simulink model "RESILIENT"  (R2018b)
settings: Solver=VariableStepAuto  StartTime=0.0  StopTime=10.0  RelTol=1e-3
undefined symbols (not defined in the file): sigbuilder_block
settings Model: Creator=lenovo  LastModifiedBy=lenovo

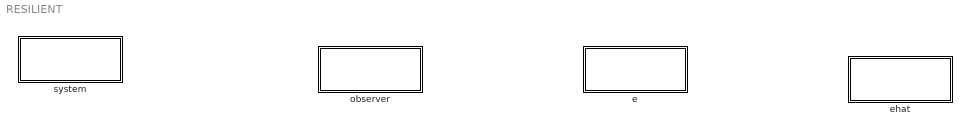
== system RESILIENT ==
  e : Subsystem
  ehat : Subsystem
  observer : Subsystem
  system : Subsystem

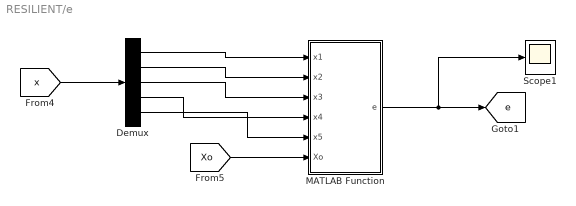
== system RESILIENT/e ==
  Demux : Demux  Outputs=5
  MATLAB Function : MATLAB Function  TreatAsAtomicUnit=on
  Scope1 : Scope
  tag scope: e=global
  wires:
  MATLAB Function/1(e) -> Scope1/1, [e]
  Demux/2 -> MATLAB Function/2(x2)
  Demux/1 -> MATLAB Function/1(x1)
  Demux/5 -> MATLAB Function/5(x5)
  [x] -> Demux/1
  Demux/4 -> MATLAB Function/4(x4)
  [Xo] -> MATLAB Function/6(Xo)
  Demux/3 -> MATLAB Function/3(x3)

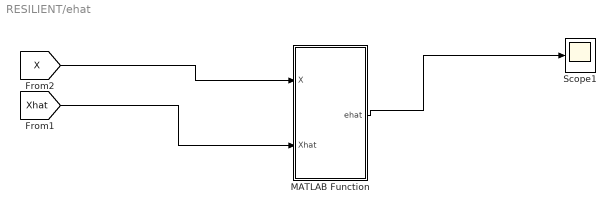
== system RESILIENT/ehat ==
  MATLAB Function : MATLAB Function  TreatAsAtomicUnit=on
  Scope1 : Scope
  wires:
  MATLAB Function/1(ehat) -> Scope1/1
  [X] -> MATLAB Function/1(X)
  [Xhat] -> MATLAB Function/2(Xhat)

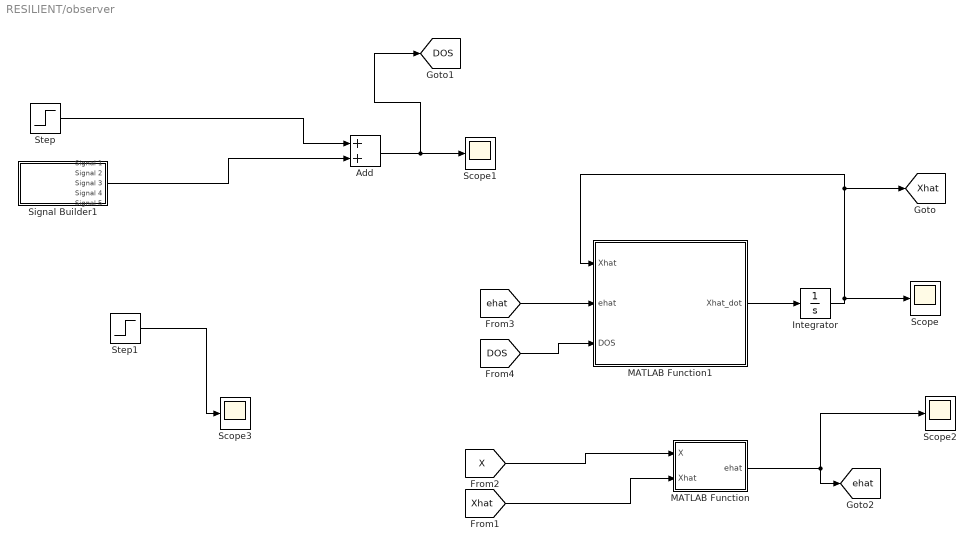
== system RESILIENT/observer ==
  Add : Sum
  Integrator : Integrator  InitialCondition=[-0.5;-1;-1.5;-2;-2.5;-3;-3.5;-4;-4.5;-5;-5.5;-6;0.5;1;1.5;2;2.5;3;3.5;4;4.5;5;5.5;6]
  MATLAB Function : MATLAB Function  TreatAsAtomicUnit=on
  MATLAB Function1 : MATLAB Function  TreatAsAtomicUnit=on
  Scope{,1..3} (4 alike) : Scope
  Signal Builder1 : Subsystem  Tag=STV Subsys  LoadFcn=sigbuilder_block('load',[5.4 30 1141.2 522.6 ]);  StartFcn=sigbuilder_block('start');  StopFcn=sigbuilder_block('stop');  ClipboardFcn=sigbuilder_block('clipboard');  mask(Sigbuilder block){tuvar=[0:10]}
      mask help: Simulink:masks:SigbuilderBlock_MD
      mask init:
      | if ~strcmp(get_param(bdroot(gcbh),'SimulationStatus'),'stopped') tuvar = sigbuilder_block('maskInit'); end
      settings: CopyFcn=sigbuilder_block('copy');  DeleteFcn=sigbuilder_block('delete');  ModelCloseFcn=sigbuilder_block('modelClose');  PreSaveFcn=sigbuilder_block('preSave');  PauseFcn=sigbuilder_block('pause');  ContinueFcn=sigbuilder_block('continue');  NameChangeFcn=sigbuilder_block('namechange');  OpenFcn=sigbuilder_block('open',[5.4 30 1141.2 522.6 ]);  CloseFcn=sigbuilder_block('close');
      mask Display: plot(0, 0, 100, 100,[2, 2, 32, 32, 2], [68, 8, 8, 68, 68],[32, 2], [38, 38], [32, 19, 2],[53, 60, 44], [32, 17, 17, 2],[16, 16, 31, 31]);txt = getActiveGroup(gcbh);text(2, 100, txt,'verticalAlignment', 'top');
  Step : Step  After=-1  SampleTime=5
  Step1 : Step  Before=1  After=0  SampleTime=5
  tag scope: DOS=global, Xhat=global, ehat=global
  wires:
  MATLAB Function1/1(Xhat_dot) -> Integrator/1
  Integrator/1 -> Scope/1, [Xhat], MATLAB Function1/1(Xhat)
  [ehat] -> MATLAB Function1/2(ehat)
  MATLAB Function/1(ehat) -> [ehat], Scope2/1
  [X] -> MATLAB Function/1(X)
  [Xhat] -> MATLAB Function/2(Xhat)
  Add/1 -> [DOS], Scope1/1
  Step/1 -> Add/1
  Signal Builder1/3(Signal 3) -> Add/2
  Step1/1 -> Scope3/1
  [DOS] -> MATLAB Function1/3(DOS)

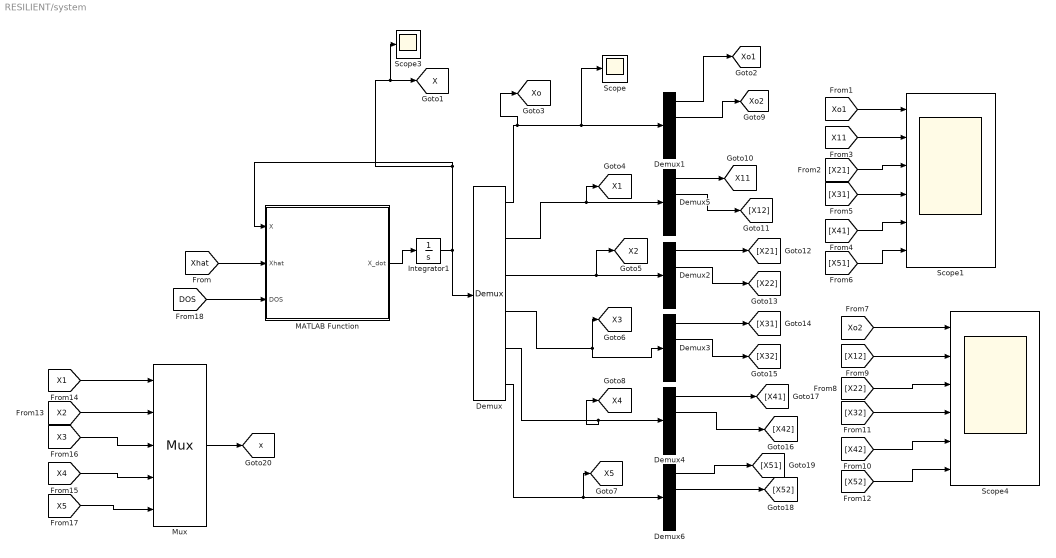
== system RESILIENT/system ==
  Demux : Demux  Outputs=6
  Demux{1..6} (6 alike) : Demux
  Integrator1 : Integrator  InitialCondition=[-0.5;-1;-1.5;-2;-2.5;-3;-3.5;-4;-4.5;-5;-5.5;-6;0.5;1;1.5;2;2.5;3;3.5;4;4.5;5;5.5;6]
  MATLAB Function : MATLAB Function  TreatAsAtomicUnit=on
  Mux : Mux  Inputs=5
  Scope : Scope
  Scope1 : Scope  NumInputPorts=6
  Scope3 : Scope
  Scope4 : Scope  NumInputPorts=6
  tag scope: X11=global, X1=global, X2=global, X3=global, X4=global, X5=global, X=global, Xo1=global, Xo2=global, Xo=global, x=global
  wires:
  Demux/2 -> [X1], Demux5/1
  Demux/3 -> [X2], Demux2/1
  Demux/1 -> [Xo], Scope/1, Demux1/1
  Demux/4 -> [X3], Demux3/1
  Demux/6 -> [X5], Demux6/1
  Demux/5 -> [X4], Demux4/1
  [Xhat] -> MATLAB Function/2(Xhat)
  MATLAB Function/1(X_dot) -> Integrator1/1
  Integrator1/1 -> MATLAB Function/1(X), Scope3/1, [X], Demux/1
  Demux1/1 -> [Xo1]
  Demux1/2 -> [Xo2]
  Demux5/1 -> [X11]
  Demux5/2 -> [X12]
  Demux2/1 -> [X21]
  Demux2/2 -> [X22]
  Demux3/1 -> [X31]
  Demux3/2 -> [X32]
  Demux4/1 -> [X41]
  Demux4/2 -> [X42]
  Demux6/1 -> [X51]
  Demux6/2 -> [X52]
  [Xo1] -> Scope1/1
  [X11] -> Scope1/2
  [X21] -> Scope1/3
  [X31] -> Scope1/4
  [X41] -> Scope1/5
  [X51] -> Scope1/6
  [X52] -> Scope4/6
  [X22] -> Scope4/3
  [X32] -> Scope4/4
  [X12] -> Scope4/2
  [X42] -> Scope4/5
  [Xo2] -> Scope4/1
  [X1] -> Mux/1
  [X2] -> Mux/2
  [X3] -> Mux/3
  [X4] -> Mux/4
  [X5] -> Mux/5
  Mux/1 -> [x]
  [DOS] -> MATLAB Function/3(DOS)

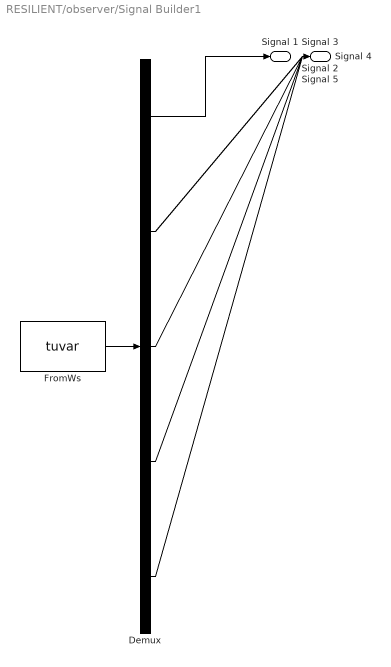
== system RESILIENT/observer/Signal Builder1 ==
  Demux : Demux  Tag=STV Demux  Outputs=5
  FromWs : FromWorkspace  Tag=STV FromWs  VariableName=tuvar  SampleTime=0
      SigBuilderData=|
      | common.afterFinalStr = 'Extrapolate'
      | common.sampleTime = 0
      | dataSet.timeRange = [0 10]
      | dataSet.name = 'Group 1'
      | sbobj.Groups.Name = 'Group 1'
      | sbobj.Groups.Signals(1).Name = 'Signal 1'
      | sbobj.Groups.Signals(1).XData = [0 4 4 6 6 10]
      | sbobj.Groups.Signals(1).YData = [0 0 1 1 0 0]
      | sbobj.Groups.Signals(2).Name = 'Signal 2'
      | sbobj.Groups.Signals(2).XData = [0 0.125 0.125 0.25 0.25 0.375 0.375 0.5 0.5 0.625 0.625 0.75 0.75 0.875 0.875 1 1 1.125 1.125 1.25 1.25 1.375 1.375 1.5 1.5 1.625 1.625 1.75 1.75 1.875 1.875 2 2 2.125 2.125 2.25 2.25 2.375 2.375 2.5 2.5 2.625 2.625 2.75 2.75 2.875 2.875 3 3 3.125 3.125 3.25 3.25 3.375 3.375 3.5 3.5 3.625 3.625 3.75 3.75 3.875 3.875 4 4 4.125 4.125 4.25 4.25 4.375 4.375 4.5 4.5 4.625 4.625 4.75 4.75 4.875 4.875 5 5 5.125 5.125 5.25 5.25 5.375 5.375 5.5 5.5 5.625 5.625 5.75 5.75 5.875 5.875 6 6 6.125 6.125 6.25 6.25 6.375 6.375 6.5 6.5 6.625 6.625 6.75 6.75 6.875 6.875 7 7 7.125 7.125 7.25 7.25 7.375 7.375 7.5 7.5 7.625 7.625 7.75 7.75 7.875 7.875 8 8 8.125 8.125 8.25 8.25 8.375 8.375 8.5 8.5 8.625 8.625 8.75 8.75 8.875 8.875 9 9 9.125 9.125 9.25 9.25 9.375 9.375 9.5 9.5 9.625 9.625 9.75 9.75 9.875 9.875 10]
      | sbobj.Groups.Signals(2).YData = [1 1 -1 -1 1 1 -1 -1 1 1 -1 -1 1 1 -1 -1 1 1 -1 -1 1 1 -1 -1 1 1 -1 -1 1 1 -1 -1 1 1 -1 -1 1 1 -1 -1 1 1 -1 -1 1 1 -1 -1 1 1 -1 -1 1 1 -1 -1 1 1 -1 -1 1 1 -1 -1 1 1 -1 -1 1 1 -1 -1 1 1 -1 -1 1 1 -1 -1 1 1 -1 -1 1 1 -1 -1 1 1 -1 -1 1 1 -1 -1 1 1 -1 -1 1 1 -1 -1 1 1 -1 -1 1 1 -1 -1 1 1 -1 -1 1 1 -1 -1 1 1 -1 -1 1 1 -1 -1 1 1 -1 -1 1 1 -1 -1 1 1 -1 -1 1 1 -1 -1 1 1 -1 -1 1 1 -1 -1 1 1 -1 -1 1 1 -1 -1]
      | sbobj.Groups.Signals(3).Name = 'Signal 3'
      | sbobj.Groups.Signals(3).XData = [0 0.16 0.333333333333 0.4 0.4 0.46 0.46 0.833333333333 1 1.005 1.005 1.3 1.3 1.8 1.8 1.9 1.9 2.4 2.4 2.55 2.55 2.625 2.785 2.83333333333 3 3.2 3.2 3.4 3.4 3.5 3.66666666667 3.83333333333 4 4 4.17 4.17 4.33333333333 4.5 4.8 4.8 4.85 4.85 5 5.16666666667 5.33333333333 5.5 5.66666666667 5.83333333333 6 6.16666666667 6.33333333333 6.5 6.66666666667 6.83333333333 7 7.16666666667 7.33333333333 7.5 7.66666666667 7.83333333333 8 8.16666666667 8.33333333333 8.5 8.66666666667 8.83333333333 9 9.16666666667 9.33333333333 9.5 9.66666666667 9.83333333333 10]
      | sbobj.Groups.Signals(3).YData = [1 1 1 1 0 0 1 1 1 1 0 0 1 1 0 0 1 1 0 0 1 1 1 1 1 1 0 0 1 1 1 1 1 0 0 1 1 1 1 0 0 1 1 1 1 1 1 1 1 1 1 1 1 1 1 1 1 1 1 1 1 1 1 1 1 1 1 1 1 1 1 1 1]
      | sbobj.Groups.Signals(4).Name = 'Signal 4'
      | sbobj.Groups.Signals(4).XData = [0 5 5 10]
      | sbobj.Groups.Signals(4).YData = [0 0 1 1]
      | sbobj.Groups.Signals(5).Name = 'Signal 5'
      | sbobj.Groups.Signals(5).XData = [0 0.45 0.45 0.5 0.5 0.95 0.95 1 1 1.45 1.45 1.5 1.5 1.95 1.95 2 2 2.45 2.45 2.5 2.5 2.95 2.95 3 3 3.45 3.45 3.5 3.5 3.95 3.95 4 4 4.45 4.45 4.5 4.5 4.95 4.95 5 5 5.45 5.45 5.5 5.5 5.95 5.95 6 6 6.45 6.45 6.5 6.5 6.95 6.95 7 7 7.45 7.45 7.5 7.5 7.95 7.95 8 8 8.45 8.45 8.5 8.5 8.95 8.95 9 9 9.45 9.45 9.5 9.5 9.95 9.95 10]
      | sbobj.Groups.Signals(5).YData = [2 2 0 0 2 2 0 0 2 2 0 0 2 2 0 0 2 2 0 0 2 2 0 0 2 2 0 0 2 2 0 0 2 2 0 0 2 2 0 0 2 2 0 0 2 2 0 0 2 2 0 0 2 2 0 0 2 2 0 0 2 2 0 0 2 2 0 0 2 2 0 0 2 2 0 0 2 2 0 0]
  Signal 1 : Outport  Tag=STV Outport
  Signal 2 : Outport  Tag=STV Outport  Port=2
  Signal 3 : Outport  Tag=STV Outport  Port=3
  Signal 4 : Outport  Tag=STV Outport  Port=4
  Signal 5 : Outport  Tag=STV Outport  Port=5
  wires:
  Demux/1 -> Signal 1/1
  FromWs/1 -> Demux/1
  Demux/2 -> Signal 2/1
  Demux/3 -> Signal 3/1
  Demux/4 -> Signal 4/1
  Demux/5 -> Signal 5/1

== matlab function RESILIENT/observer/MATLAB Function1 ==
  data: Xhat input; Xhat_dot output; ehat input; DOS input
function Xhat_dot = X(Xhat,ehat,DOS)
A=[0 1 0 0;-48.6 -1.26 48.6 0;0 0 0 10; 1.95 0 -1.95 0];
B=[0;21.6;0;0];
C=[1 0 1 -1;0 1 0 0];
c=2;
teta=5;
H=[3.0849 0.6931;2.4258 34.9384;7.0235 3.5334;.54 1.8007];
R=[-0.9886 0.0381;0 -1; -1.0405 .0402;-1.0291 0.0783]


N=6;



%L=[0 0 0 0 0 0;-1 2 0 0 0 -1;-1 -1 2 0 0 0;0 -1 0 1 0 0;0 0 -1 0 1 0;0 0 -1 -1 -1 3];


LO=[0 0 0 0 0 0;-1 1 0 0 0 0;0 -1 1 0 0 0;0 0 0 0 0 0;0 0 -1 0 1 0;0 0 0 -1 -1 2];
L=[0 0 0 0 0 0;-1 2-DOS 0 0 0 -1+DOS;-1+DOS -1 2-DOS 0 0 0;0 -1+DOS 0 1-DOS 0 0;0 0 -1 0 1 0;0 0 -1+DOS -1 -1 3-DOS];
LC=[0 0 0 0 0 0;0 0 0 0 0 0;-1 -1 2 0 0 0;0 -1 0 1 0 0;0 0 0 0 0 0;0 0 -1 -1 -1 3];



K=[79.1094 5.2218 -29.6598 163.9093];




A0=kron(eye(N),A);
z1=kron(L,B*K);
z2=kron(L,H*C);
 

Xhat_dot= (A0-c*z1)*Xhat+teta*(z2*ehat);

== matlab function RESILIENT/system/MATLAB Function ==
  data: X input; X_dot output; Xhat input; DOS input
function X_dot = X(X,Xhat,DOS)
A=[0 1 0 0;-48.6 -1.26 48.6 0;0 0 0 10; 1.95 0 -1.95 0];
B=[0;21.6;0;0];
C=[1 0 1 -1;0 1 0 0];
c=2;

N=6;

L=[0 0 0 0 0 0;-1 2 0 0 0 -1;-1 -1 2 0 0 0;0 -1 0 1 0 0;0 0 -1 0 1 0;0 0 -1 -1 -1 3];
%Lo=[0 0 0 0 0 0;-1 1 0 0 0 0;0 -1 1 0 0 0;0 0 0 0 0 0;0 0 -1 0 1 0;0 0 0 -1 -1 2];
LC=[0 0 0 0 0 0;0 0 0 0 0 0;-1 -1 2 0 0 0;0 -1 0 1 0 0;0 0 0 0 0 0;0 0 -1 -1 -1 3];

%L=[0 0 0 0 0 0;-1+DOS 2-2*DOS 0 0 0 -1+DOS;-1 -1 2 0 0 0;0 -1 0 1 0 0;0 0 -1+DOS 0 1-DOS 0;0 0 -1 -1 -1 3];
K=[79.1094 5.2218 -29.6598 163.9093];



A0=kron(eye(N),A);
z1=kron(L,B*K);
 


X_dot= A0*X-c*(z1*Xhat);

== matlab function RESILIENT/e/MATLAB Function ==
  data: x1 input; x2 input; x3 input; x4 input; x5 input; e output; Xo input
function e = fcn(x1,x2,x3,x4,x5,Xo)

e =0.2* norm(x1-Xo+x2-Xo+x3-Xo+x4-Xo+x5-Xo);

== matlab function RESILIENT/ehat/MATLAB Function ==
  data: X input; Xhat input; ehat output
function ehat = fcn(X,Xhat)

ehat = norm(X-Xhat);

== matlab function RESILIENT/observer/MATLAB Function ==
  data: X input; ehat output; Xhat input
function ehat = fcn(X,Xhat)

ehat =( X-Xhat);
